simulink model "control_loop_model_ziegler_nichols"  (R2025b)
settings: Solver=FixedStepAuto  StartTime=0.0  StopTime=10000  FixedStep=1  RelTol=1e-3
undefined symbols (not defined in the file): K, T1, T_offset, Tt
libraries: simulink x4
settings Model: Creator=robin  LastModifiedBy=robin

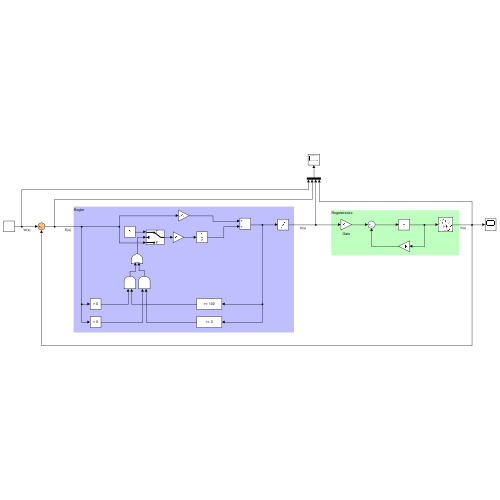
[thumbnail: Simulink's stored preview of the top-level diagram]
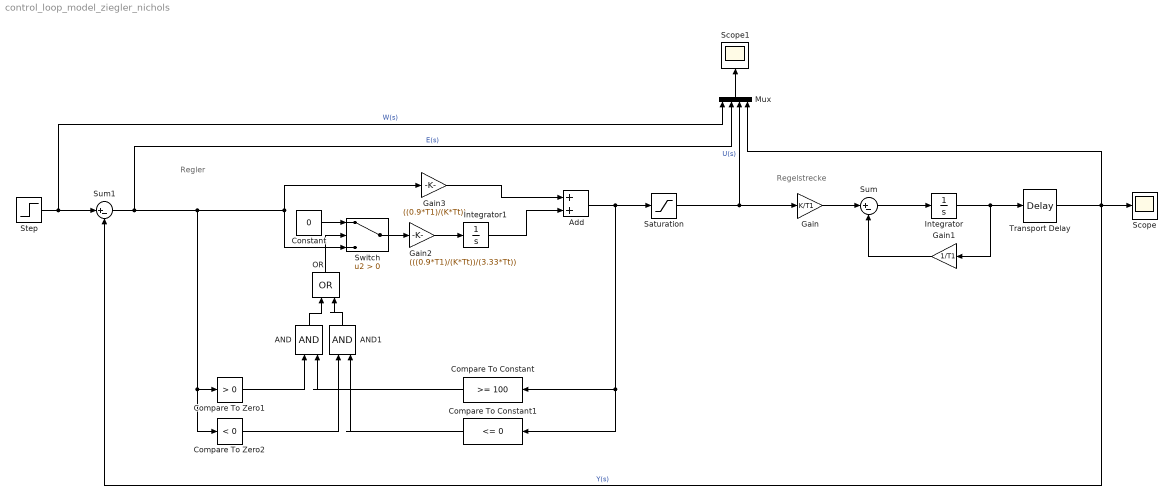
== system control_loop_model_ziegler_nichols ==
  note: Regler
  note: Regelstrecke
  AND : Logic  IconShape=distinctive  AllPortsSameDT=off  OutDataTypeStr=boolean
  AND1 : Logic  IconShape=distinctive  AllPortsSameDT=off  OutDataTypeStr=boolean
  Add : Sum
  Compare To Constant : simulink/Logic and Bit Operations/Compare To Constant  relop=>=  const=100  OutDataTypeStr=boolean
  Compare To Constant1 : simulink/Logic and Bit Operations/Compare To Constant  relop=<=  const=0  OutDataTypeStr=boolean
  Compare To Zero1 : simulink/Logic and Bit Operations/Compare To Zero  relop=>  OutDataTypeStr=boolean
  Compare To Zero2 : simulink/Logic and Bit Operations/Compare To Zero  relop=<  OutDataTypeStr=boolean
  Constant : Constant  Value=0
  Gain : Gain  Gain=K/T1
  Gain1 : Gain  Gain=1/T1
  Gain2 : Gain  Gain=(((0.9*T1)/(K*Tt))/(3.33*Tt))
  Gain3 : Gain  Gain=((0.9*T1)/(K*Tt))
  Integrator : Integrator  InitialCondition=T_offset
  Integrator1 : Integrator
  Mux : Mux
  OR : Logic  Operator=OR  IconShape=distinctive  AllPortsSameDT=off  OutDataTypeStr=boolean
  Saturation : Saturate  UpperLimit=100  LowerLimit=0
  Scope : Scope
      settings: ActiveDisplayYMinimum=1888.1958650332126  ActiveDisplayYMaximum=7627.7166667025294
  Scope1 : Scope
      settings: ActiveDisplayYMinimum=-3653.0143498935763  ActiveDisplayYMaximum=8243.4066905832842
  Step : Step  After=7000  SampleTime=0
  Sum : Sum  Inputs=|+-
  Sum1 : Sum  Inputs=|+-
  Switch : Switch  Criteria=u2 > Threshold  SaturateOnIntegerOverflow=off  InputSameDT=off
  Transport Delay : TransportDelay  DelayTime=Tt  InitialOutput=T_offset
  wires:
  Gain1/1 -> Sum/2
  Integrator/1 -> Transport Delay/1, Gain1/1
  Sum/1 -> Integrator/1
  Gain/1 -> Sum/1
  Switch/1 -> Gain2/1
  AND1/1 -> OR/2
  Gain2/1 -> Integrator1/1
  Sum1/1 -> Mux/2, Switch/3, Gain3/1, Compare To Zero2/1, Compare To Zero1/1  "E(s)"
  Constant/1 -> Switch/1
  AND/1 -> OR/1
  Compare To Constant1/1 -> AND1/2
  OR/1 -> Switch/2
  Integrator1/1 -> Add/2
  Compare To Constant/1 -> AND/2
  Add/1 -> Saturation/1, Compare To Constant1/1, Compare To Constant/1
  Gain3/1 -> Add/1
  Compare To Zero2/1 -> AND1/1
  Compare To Zero1/1 -> AND/1
  Step/1 -> Mux/1, Sum1/1  "W(s)"
  Saturation/1 -> Gain/1, Mux/3  "U(s)"
  Mux/1 -> Scope1/1
  Transport Delay/1 -> Mux/4, Sum1/2, Scope/1  "Y(s)"
